simulink model "structure_env"  (R2026b)
settings: Solver=VariableStepAuto
undefined symbols (not defined in the file or in its folder): P, Ts
libraries: simulink x3
settings Model: Creator=aomar  LastModifiedBy=aomar

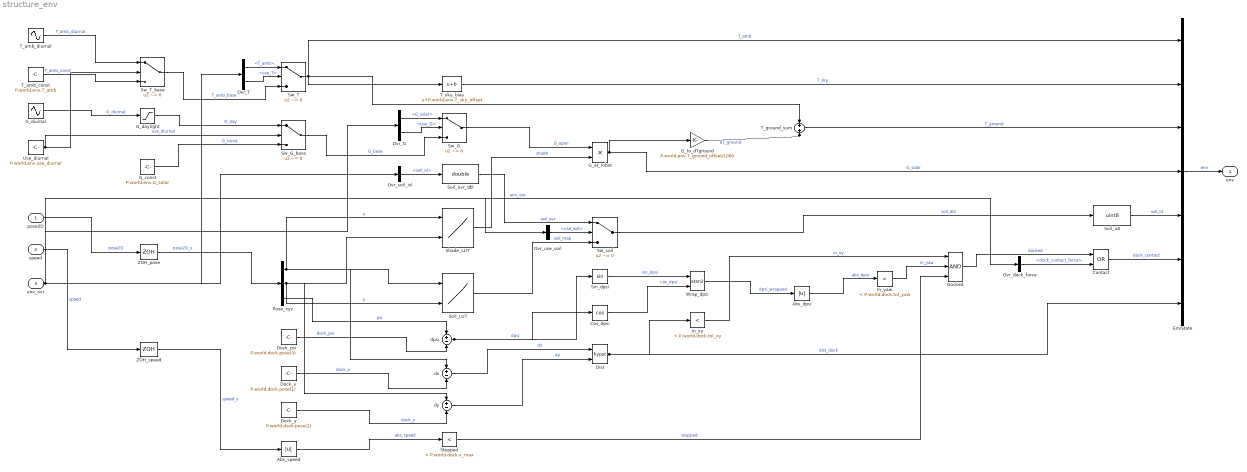
== system structure_env ==
  pose2D : Inport  OutDataTypeStr=double  PortDimensions=3  SampleTime=0
  speed : Inport  Port=2  OutDataTypeStr=double  PortDimensions=1  SampleTime=0
  env_ovr : Inport  Port=3  OutDataTypeStr=Bus: Bus_EnvOverride  SampleTime=Ts.env
  Abs_dpsi : Abs  SaturateOnIntegerOverflow=off
  Abs_speed : Abs  SaturateOnIntegerOverflow=off
  Contact : Logic  Operator=OR  AllPortsSameDT=off  OutDataTypeStr=boolean
  Cos_dpsi : Trigonometry  Operator=cos
  Dist : Math  Operator=hypot
  Dock_psi : Constant  Value=P.world.dock.pose(3)
  Dock_x : Constant  Value=P.world.dock.pose(1)
  Dock_y : Constant  Value=P.world.dock.pose(2)
  Docked : Logic  Inputs=3  AllPortsSameDT=off  OutDataTypeStr=boolean
  EnvState : BusCreator  Inputs=7  OutDataTypeStr=Bus: Bus_EnvState  NonVirtualBus=on
  G_at_robot : Product
  G_const : Constant  Value=P.world.env.G_solar
  G_daylight : Saturate  UpperLimit=inf  LowerLimit=0
  G_diurnal : Sin  Amplitude=P.world.env.diurnal.G_pk  Frequency=2*pi/86400  Phase=2*pi*(P.world.env.diurnal.t0_hour - 6)/24  SampleTime=Ts.env
  G_to_dTground : Gain  Gain=P.world.env.T_ground_offset/1000
  In_xy : simulink/Logic and Bit Operations/Compare To Constant  relop=<  const=P.world.dock.tol_xy  OutDataTypeStr=boolean
  In_yaw : simulink/Logic and Bit Operations/Compare To Constant  relop=<  const=P.world.dock.tol_yaw  OutDataTypeStr=boolean
  Ovr_G : BusSelector  OutputSignals=G_solar,use_G
  Ovr_T : BusSelector  OutputSignals=T_amb,use_T
  Ovr_dock_force : BusSelector  OutputSignals=dock_contact_force
  Ovr_soil_id : BusSelector  OutputSignals=soil_id
  Ovr_use_soil : BusSelector  OutputSignals=use_soil
  Pose_xyz : Demux  Outputs=3
  Shade_LUT : Lookup_n-D  BreakpointsForDimension1=P.world.terrain.xE  BreakpointsForDimension2=P.world.terrain.yN  IndexSearchMethod=Evenly spaced points  Table=P.world.shade  ExtrapMethod=Clip  InternalRulePriority=Speed  RndMeth=Simplest
      settings: InputPortMap=u0,u1
  Sin_dpsi : Trigonometry
  Soil_LUT : Lookup_n-D  BreakpointsForDimension1=P.world.terrain.xE  BreakpointsForDimension2=P.world.terrain.yN  IndexSearchMethod=Evenly spaced points  Table=P.world.soilId  InterpMethod=Nearest  ExtrapMethod=Clip  InternalRulePriority=Speed  RndMeth=Simplest
      settings: InputPortMap=u0,u1
  Soil_ovr_dbl : DataTypeConversion  OutDataTypeStr=double  SaturateOnIntegerOverflow=off  RndMeth=Floor
  Soil_u8 : DataTypeConversion  OutDataTypeStr=uint8  RndMeth=Nearest
  Stopped : simulink/Logic and Bit Operations/Compare To Constant  relop=<  const=P.world.dock.v_max  OutDataTypeStr=boolean
  Sw_G : Switch  Criteria=u2 ~= 0  SaturateOnIntegerOverflow=off  InputSameDT=off
  Sw_G_base : Switch  Criteria=u2 ~= 0  SaturateOnIntegerOverflow=off  InputSameDT=off
  Sw_T : Switch  Criteria=u2 ~= 0  SaturateOnIntegerOverflow=off  InputSameDT=off
  Sw_T_base : Switch  Criteria=u2 ~= 0  SaturateOnIntegerOverflow=off  InputSameDT=off
  Sw_soil : Switch  Criteria=u2 ~= 0  SaturateOnIntegerOverflow=off  InputSameDT=off
  T_amb_const : Constant  Value=P.world.env.T_amb
  T_amb_diurnal : Sin  Amplitude=P.world.env.diurnal.T_amp  Bias=P.world.env.diurnal.T_mean  Frequency=2*pi/86400  Phase=2*pi*(P.world.env.diurnal.t0_hour - P.world.env.diurnal.h_peak + 6)/24  SampleTime=Ts.env
  T_ground_sum : Sum
  T_sky_bias : Bias  Bias=P.world.env.T_sky_offset  SaturateOnIntegerOverflow=off
  Use_diurnal : Constant  Value=P.world.env.use_diurnal
  Wrap_dpsi : Trigonometry  Operator=atan2
  ZOH_pose : ZeroOrderHold  SampleTime=Ts.env
  ZOH_speed : ZeroOrderHold  SampleTime=Ts.env
  dpsi : Sum  Inputs=+-
  dx : Sum  Inputs=+-
  dy : Sum  Inputs=+-
  env : Outport  OutDataTypeStr=Bus: Bus_EnvState  SampleTime=Ts.env
  wires:
  T_amb_diurnal/1 -> Sw_T_base/1  "T_amb_diurnal"
  T_amb_const/1 -> Sw_T_base/3  "T_amb_const"
  G_diurnal/1 -> G_daylight/1  "G_diurnal"
  Use_diurnal/1 -> Sw_T_base/2, Sw_G_base/2  "use_diurnal"
  pose2D/1 -> ZOH_pose/1  "pose2D"
  speed/1 -> ZOH_speed/1  "speed"
  env_ovr/1 -> Ovr_T/1, Ovr_G/1, Ovr_soil_id/1, Ovr_use_soil/1, Ovr_dock_force/1  "env_ovr"
  G_daylight/1 -> Sw_G_base/1  "G_day"
  G_const/1 -> Sw_G_base/3  "G_const"
  ZOH_pose/1 -> Pose_xyz/1  "pose2D_s"
  ZOH_speed/1 -> Abs_speed/1  "speed_s"
  Sw_T_base/1 -> Sw_T/3  "T_amb_base"
  Ovr_T/1 -> Sw_T/1  "<T_amb>"
  Ovr_T/2 -> Sw_T/2  "<use_T>"
  Pose_xyz/3 -> dpsi/1  "psi"
  Dock_psi/1 -> dpsi/2  "dock_psi"
  Dock_x/1 -> dx/2  "dock_x"
  Dock_y/1 -> dy/2  "dock_y"
  Abs_speed/1 -> Stopped/1  "abs_speed"
  Sw_T/1 -> T_ground_sum/1, EnvState/1, T_sky_bias/1  "T_amb"
  Sw_G_base/1 -> Sw_G/3  "G_base"
  Ovr_G/1 -> Sw_G/1  "<G_solar>"
  Ovr_G/2 -> Sw_G/2  "<use_G>"
  Ovr_soil_id/1 -> Soil_ovr_dbl/1  "<soil_id>"
  dpsi/1 -> Sin_dpsi/1, Cos_dpsi/1  "dpsi"
  dx/1 -> Dist/1  "dx"
  dy/1 -> Dist/2  "dy"
  Stopped/1 -> Docked/3  "stopped"
  T_sky_bias/1 -> EnvState/2  "T_sky"
  Sw_G/1 -> G_at_robot/1  "G_open"
  Shade_LUT/1 -> G_at_robot/2  "shade"
  Soil_LUT/1 -> Sw_soil/3  "soil_map"
  Soil_ovr_dbl/1 -> Sw_soil/1  "soil_ovr"
  Ovr_use_soil/1 -> Sw_soil/2  "<use_soil>"
  G_at_robot/1 -> EnvState/4, G_to_dTground/1  "G_solar"
  Sin_dpsi/1 -> Wrap_dpsi/1  "sin_dpsi"
  Cos_dpsi/1 -> Wrap_dpsi/2  "cos_dpsi"
  Dist/1 -> EnvState/7, In_xy/1  "dist_dock"
  Sw_soil/1 -> Soil_u8/1  "soil_dbl"
  G_to_dTground/1 -> T_ground_sum/2  "dT_ground"
  Wrap_dpsi/1 -> Abs_dpsi/1  "dpsi_wrapped"
  In_xy/1 -> Docked/1  "in_xy"
  T_ground_sum/1 -> EnvState/3  "T_ground"
  Abs_dpsi/1 -> In_yaw/1  "abs_dpsi"
  In_yaw/1 -> Docked/2  "in_yaw"
  Docked/1 -> Contact/1  "docked"
  Ovr_dock_force/1 -> Contact/2  "<dock_contact_force>"
  Contact/1 -> EnvState/6  "dock_contact"
  Soil_u8/1 -> EnvState/5  "soil_id"
  EnvState/1 -> env/1  "env"
  Pose_xyz/1 -> Soil_LUT/1, dx/1, Shade_LUT/1  "x"
  Pose_xyz/2 -> dy/1, Shade_LUT/2, Soil_LUT/2  "y"
